simulink model "XFLUID02_reference"  (R2025a)
settings: Solver=ode23t  StartTime=0  StopTime=1.5  MaxStep=0.001  RelTol=1e-3  EnableMultiTasking=on
model workspace (MAT data in the model file):
  TRP_Par : object (value not decoded)
  fault_cylinder = 2
  inlet_area_factor = 1
  output_pressure_bar = 7
  pOutMeas_data = [7; 7]
  pOutMeas_time = [0; 1.5]
  pOut_Init_WKSP = 7
  pump_speed_rpm = 958
  seal_leak_fraction = 0
  speed_step_fraction = 0.08
  speed_step_time = 0.72
symbols that are objects in the model workspace (value not decoded): TRP_Par
undefined symbols (not defined in the file): Plunger, sm_pump_triplex_lib, smiData, X, Y, Z
libraries: sm_lib x133, fl_lib x62, nesl_utility x24, SimscapeFluids_lib x15, simulink x10, ee_lib x2
(part 5 of 7)

== system XFLUID02_reference/Pump/Plunger 1/Flow Out ==
  Gain : Gain  Gain=0.01/5
  Hydraulic Flow Rate Sensor : fl_lib/Isothermal Liquid/Sensors/Flow Rate Sensor (IL)  sensor_type=3
      settings: InternalSimscapePortConfiguration="{\"Bottom\":[],\"Left\":[{\"id\":\"A\",\"label\":\"A\",\"type\":\"foundation.isothermal_liquid.isothermal_liquid\"}],\"Right\":[{\"id\":\"B\",\"label\":\"B\",\"type\":\"foundation.isothermal_liquid.isothermal_liquid\"},{\"id\":\"M\",\"label\":\"M\",\"type\":\"output\"},{\"id\":\"V\",\"label\":\"V\",\"type\":\"output\"}],\"Top\":[]}"
      settings: LibrarySourceBlock=|
      | fl_lib/Hydraulic/Hydraulic Sensors/Hydraulic Flow Rate
      | Sensor
  Log_plunger1_flow : ToWorkspace  VariableName=plunger1_flow  SaveFormat=Timeseries  SampleTime=-1
  Lowpass Filter : TransferFcn  Denominator=[1/(2*pi*100) 1]
  PS Terminator : fl_lib/Physical Signals/Sinks/PS Terminator
  PS-Simulink Converter : nesl_utility/PS-Simulink Converter  PhysicalDomain=network_engine_domain  SubClassName=ps_output  LeftPortType=input  RightPortType=output  PseudoPeriodic=off  Frequencies=[]  VectorFormat=1-D array  Unit=lpm  AffineConversion=off
  Saturation : Saturate  UpperLimit=5  LowerLimit=0  ZeroCross=off
  A : PMIOPort  Side=Left
  B : PMIOPort  Port=2  Side=Right
  q : Outport  VectorParamsAs1DForOutWhenUnconnected=off
  wires:
  PS-Simulink Converter/1 -> Saturation/1, Log_plunger1_flow/1
  Saturation/1 -> Gain/1
  Gain/1 -> Lowpass Filter/1
  Lowpass Filter/1 -> q/1
  connections:
  PS Terminator/LConn1 -- Hydraulic Flow Rate Sensor/RConn2
  B/RConn1 -- Hydraulic Flow Rate Sensor/RConn1
  A/RConn1 -- Hydraulic Flow Rate Sensor/LConn1
  PS-Simulink Converter/LConn1 -- Hydraulic Flow Rate Sensor/RConn3

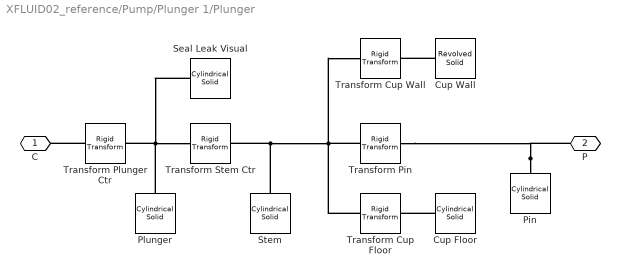
== system XFLUID02_reference/Pump/Plunger 1/Plunger ==
  Cup Floor : sm_lib/Body Elements/Cylindrical Solid  CylinderRadius=cup_rad_out-cup_thk  CylinderRadiusUnits=m  CylinderLength=cup_thk  CylinderLengthUnits=m  ExportEntireGeometry=off  InertiaType=CalculateFromGeometry  BasedOnType=Density  Density=plg_rho  DensityUnits=kg/m^3  Mass=1  MassUnits=kg  CenterOfMass=[0 0 0]  CenterOfMassUnits=m  MomentsOfInertia=[1 1 1]  MomentsOfInertiaUnits=kg*m^2  ProductsOfInertia=[1 1 1]  ProductsOfInertiaUnits=kg*m^2  GraphicType=FromGeometry  MarkerShape=Sphere  MarkerSize=10  GraphicVisPropType=SimpleVisualProperties  GraphicDiffuseColor=plg_clr  GraphicOpacity=plg_opc  GraphicSpecularColor=[0.5 0.5 0.5 1.0]  GraphicAmbientColor=[0.15 0.15 0.15 1.0]  GraphicEmissiveColor=[0.0 0.0 0.0 1.0]  GraphicShininess=75  DoExposeReferenceFrame=on  SerializedFrames=<Frames/>
  Cup Wall : sm_lib/Body Elements/Revolved Solid  RevolutionCrossSection=cup_xc_rev  RevolutionCrossSectionUnits=m  RevolutionExtent=Full  RevolutionAngle=180  RevolutionAngleUnits=deg  ExportConvexHullGeometry=off  InertiaType=CalculateFromGeometry  BasedOnType=Density  Density=plg_rho  DensityUnits=kg/m^3  Mass=1  MassUnits=kg  CenterOfMass=[0 0 0]  CenterOfMassUnits=m  MomentsOfInertia=[1 1 1]  MomentsOfInertiaUnits=kg*m^2  ProductsOfInertia=[1 1 1]  ProductsOfInertiaUnits=kg*m^2  GraphicType=FromGeometry  MarkerShape=Sphere  MarkerSize=10  GraphicVisPropType=SimpleVisualProperties  GraphicDiffuseColor=plg_clr  GraphicOpacity=plg_opc  GraphicSpecularColor=[0.5 0.5 0.5 1.0]  GraphicAmbientColor=[0.15 0.15 0.15 1.0]  GraphicEmissiveColor=[0.0 0.0 0.0 1.0]  GraphicShininess=75  DoExposeReferenceFrame=on  SerializedFrames=<Frames/>
  Pin : sm_lib/Body Elements/Cylindrical Solid  CylinderRadius=pin_rad  CylinderRadiusUnits=m  CylinderLength=pin_len  CylinderLengthUnits=m  ExportEntireGeometry=off  InertiaType=CalculateFromGeometry  BasedOnType=Density  Density=plg_rho  DensityUnits=kg/m^3  Mass=1  MassUnits=kg  CenterOfMass=[0 0 0]  CenterOfMassUnits=m  MomentsOfInertia=[1 1 1]  MomentsOfInertiaUnits=kg*m^2  ProductsOfInertia=[1 1 1]  ProductsOfInertiaUnits=kg*m^2  GraphicType=FromGeometry  MarkerShape=Sphere  MarkerSize=10  GraphicVisPropType=SimpleVisualProperties  GraphicDiffuseColor=conrod_clr*0.5  GraphicOpacity=conrod_opc  GraphicSpecularColor=[0.5 0.5 0.5 1.0]  GraphicAmbientColor=[0.15 0.15 0.15 1.0]  GraphicEmissiveColor=[0.0 0.0 0.0 1.0]  GraphicShininess=75  DoExposeReferenceFrame=on  SerializedFrames=<Frames/>
  Plunger : sm_lib/Body Elements/Cylindrical Solid  CylinderRadius=plgB_rad  CylinderRadiusUnits=m  CylinderLength=plgB_len  CylinderLengthUnits=m  ExportEntireGeometry=off  InertiaType=CalculateFromGeometry  BasedOnType=Density  Density=plg_rho  DensityUnits=kg/m^3  Mass=1  MassUnits=kg  CenterOfMass=[0 0 0]  CenterOfMassUnits=m  MomentsOfInertia=[1 1 1]  MomentsOfInertiaUnits=kg*m^2  ProductsOfInertia=[1 1 1]  ProductsOfInertiaUnits=kg*m^2  GraphicType=FromGeometry  MarkerShape=Sphere  MarkerSize=10  GraphicVisPropType=SimpleVisualProperties  GraphicDiffuseColor=plg_clr  GraphicOpacity=plg_opc  GraphicSpecularColor=[0.5 0.5 0.5 1.0]  GraphicAmbientColor=[0.15 0.15 0.15 1.0]  GraphicEmissiveColor=[0.0 0.0 0.0 1.0]  GraphicShininess=75  DoExposeReferenceFrame=on  SerializedFrames=<Frames/>
  Seal Leak Visual : sm_lib/Body Elements/Cylindrical Solid  CylinderRadius=seal_leak_vis_rad  CylinderRadiusUnits=m  CylinderLength=seal_leak_vis_len  CylinderLengthUnits=m  ExportEntireGeometry=off  InertiaType=CalculateFromGeometry  BasedOnType=Density  Density=0.0001  DensityUnits=kg/m^3  Mass=1  MassUnits=kg  CenterOfMass=[0 0 0]  CenterOfMassUnits=m  MomentsOfInertia=[1 1 1]  MomentsOfInertiaUnits=kg*m^2  ProductsOfInertia=[1 1 1]  ProductsOfInertiaUnits=kg*m^2  GraphicType=FromGeometry  MarkerShape=Sphere  MarkerSize=10  GraphicVisPropType=SimpleVisualProperties  GraphicDiffuseColor=seal_leak_vis_clr  GraphicOpacity=seal_leak_vis_opc  GraphicSpecularColor=[0.5 0.5 0.5 1.0]  GraphicAmbientColor=[0.15 0.15 0.15 1.0]  GraphicEmissiveColor=[0.0 0.0 0.0 1.0]  GraphicShininess=75  DoExposeReferenceFrame=on  SerializedFrames=<Frames/>
  Stem : sm_lib/Body Elements/Cylindrical Solid  CylinderRadius=stem_rad  CylinderRadiusUnits=m  CylinderLength=stem_len  CylinderLengthUnits=m  ExportEntireGeometry=off  InertiaType=CalculateFromGeometry  BasedOnType=Density  Density=plg_rho  DensityUnits=kg/m^3  Mass=1  MassUnits=kg  CenterOfMass=[0 0 0]  CenterOfMassUnits=m  MomentsOfInertia=[1 1 1]  MomentsOfInertiaUnits=kg*m^2  ProductsOfInertia=[1 1 1]  ProductsOfInertiaUnits=kg*m^2  GraphicType=FromGeometry  MarkerShape=Sphere  MarkerSize=10  GraphicVisPropType=SimpleVisualProperties  GraphicDiffuseColor=plg_clr  GraphicOpacity=plg_opc  GraphicSpecularColor=[0.5 0.5 0.5 1.0]  GraphicAmbientColor=[0.15 0.15 0.15 1.0]  GraphicEmissiveColor=[0.0 0.0 0.0 1.0]  GraphicShininess=75  DoExposeReferenceFrame=on  SerializedFrames=<Frames/>
  Transform Cup Floor : sm_lib/Frames and Transforms/Rigid Transform  RotationMethod=None  FollAlignAxisA=+X  BaseAlignAxisA=+Y  FollAlignAxisB=+Y  BaseAlignAxisB=+Z  RotationStandardAxis=+Z  RotationAngle=0.0  RotationAngleUnits=deg  RotationArbitraryAxis=[0 0 1]  RotationSequenceAxes=FollowerAxes  RotationSequence=XYX  RotationSequenceAngles=[0 0 0]  RotationSequenceAnglesUnits=deg  RotationMatrix=[1 0 0; 0 1 0; 0 0 1]  Quaternion=[1 0 0 0]  TranslationMethod=StandardAxis  TranslationCartesianOffset=[0 0 0]  TranslationCartesianOffsetUnits=m  TranslationStandardAxis=+Z  TranslationStandardOffset=stem_len/2+cup_thk/2  TranslationStandardOffsetUnits=m  TranslationROffset=0  TranslationROffsetUnits=m  TranslationThetaOffset=0  TranslationThetaOffsetUnits=deg  TranslationZOffset=0  TranslationZOffsetUnits=m
  Transform Cup Wall : sm_lib/Frames and Transforms/Rigid Transform  RotationMethod=None  FollAlignAxisA=+X  BaseAlignAxisA=+Y  FollAlignAxisB=+Y  BaseAlignAxisB=+Z  RotationStandardAxis=+Z  RotationAngle=0.0  RotationAngleUnits=deg  RotationArbitraryAxis=[0 0 1]  RotationSequenceAxes=FollowerAxes  RotationSequence=XYX  RotationSequenceAngles=[0 0 0]  RotationSequenceAnglesUnits=deg  RotationMatrix=[1 0 0; 0 1 0; 0 0 1]  Quaternion=[1 0 0 0]  TranslationMethod=StandardAxis  TranslationCartesianOffset=[0 0 0]  TranslationCartesianOffsetUnits=m  TranslationStandardAxis=+Z  TranslationStandardOffset=stem_len/2+cup_len/2  TranslationStandardOffsetUnits=m  TranslationROffset=0  TranslationROffsetUnits=m  TranslationThetaOffset=0  TranslationThetaOffsetUnits=deg  TranslationZOffset=0  TranslationZOffsetUnits=m
  Transform Plunger Ctr : sm_lib/Frames and Transforms/Rigid Transform  RotationMethod=None  FollAlignAxisA=+X  BaseAlignAxisA=+Y  FollAlignAxisB=+Y  BaseAlignAxisB=+Z  RotationStandardAxis=+Z  RotationAngle=0.0  RotationAngleUnits=deg  RotationArbitraryAxis=[0 0 1]  RotationSequenceAxes=FollowerAxes  RotationSequence=XYX  RotationSequenceAngles=[0 0 0]  RotationSequenceAnglesUnits=deg  RotationMatrix=[1 0 0; 0 1 0; 0 0 1]  Quaternion=[1 0 0 0]  TranslationMethod=StandardAxis  TranslationCartesianOffset=[0 0 0]  TranslationCartesianOffsetUnits=m  TranslationStandardAxis=+Z  TranslationStandardOffset=plgB_len/2  TranslationStandardOffsetUnits=m  TranslationROffset=0  TranslationROffsetUnits=m  TranslationThetaOffset=0  TranslationThetaOffsetUnits=deg  TranslationZOffset=0  TranslationZOffsetUnits=m
  Transform Stem Ctr : sm_lib/Frames and Transforms/Rigid Transform  RotationMethod=None  FollAlignAxisA=+X  BaseAlignAxisA=+Y  FollAlignAxisB=+Y  BaseAlignAxisB=+Z  RotationStandardAxis=+Z  RotationAngle=0.0  RotationAngleUnits=deg  RotationArbitraryAxis=[0 0 1]  RotationSequenceAxes=FollowerAxes  RotationSequence=XYX  RotationSequenceAngles=[0 0 0]  RotationSequenceAnglesUnits=deg  RotationMatrix=[1 0 0; 0 1 0; 0 0 1]  Quaternion=[1 0 0 0]  TranslationMethod=StandardAxis  TranslationCartesianOffset=[0 0 0]  TranslationCartesianOffsetUnits=m  TranslationStandardAxis=+Z  TranslationStandardOffset=plgB_len/2+stem_len/2  TranslationStandardOffsetUnits=m  TranslationROffset=0  TranslationROffsetUnits=m  TranslationThetaOffset=0  TranslationThetaOffsetUnits=deg  TranslationZOffset=0  TranslationZOffsetUnits=m
  Transform Pin : sm_lib/Frames and Transforms/Rigid Transform  RotationMethod=StandardAxis  FollAlignAxisA=+X  BaseAlignAxisA=+Y  FollAlignAxisB=+Y  BaseAlignAxisB=+Z  RotationStandardAxis=+Y  RotationAngle=90  RotationAngleUnits=deg  RotationArbitraryAxis=[0 0 1]  RotationSequenceAxes=FollowerAxes  RotationSequence=XYX  RotationSequenceAngles=[0 0 0]  RotationSequenceAnglesUnits=deg  RotationMatrix=[1 0 0; 0 1 0; 0 0 1]  Quaternion=[1 0 0 0]  TranslationMethod=StandardAxis  TranslationCartesianOffset=[0 0 0]  TranslationCartesianOffsetUnits=m  TranslationStandardAxis=+Z  TranslationStandardOffset=stem_len/2+cup_pinOffset  TranslationStandardOffsetUnits=m  TranslationROffset=0  TranslationROffsetUnits=m  TranslationThetaOffset=0  TranslationThetaOffsetUnits=deg  TranslationZOffset=0  TranslationZOffsetUnits=m
  C : PMIOPort  Side=Left
  P : PMIOPort  Port=2  Side=Right
  connections:
  Pin/RConn1 -- P/RConn1 -- Transform Pin/RConn1
  Cup Wall/RConn1 -- Transform Cup Wall/RConn1
  Cup Floor/RConn1 -- Transform Cup Floor/RConn1
  Plunger/RConn1 -- Transform Stem Ctr/LConn1 -- Seal Leak Visual/RConn1 -- Transform Plunger Ctr/RConn1
  Transform Plunger Ctr/LConn1 -- C/RConn1
  Stem/RConn1 -- Transform Cup Floor/LConn1 -- Transform Pin/LConn1 -- Transform Cup Wall/LConn1 -- Transform Stem Ctr/RConn1

== system XFLUID02_reference/Pump/Plunger 1/Rod ==
  Ring Pin : sm_lib/Body Elements/Revolved Solid  RevolutionCrossSection=conrod_ringP_xc_rev  RevolutionCrossSectionUnits=m  RevolutionExtent=Full  RevolutionAngle=180  RevolutionAngleUnits=deg  ExportConvexHullGeometry=off  InertiaType=CalculateFromGeometry  BasedOnType=Density  Density=conrod_rho  DensityUnits=kg/m^3  Mass=1  MassUnits=kg  CenterOfMass=[0 0 0]  CenterOfMassUnits=m  MomentsOfInertia=[1 1 1]  MomentsOfInertiaUnits=kg*m^2  ProductsOfInertia=[1 1 1]  ProductsOfInertiaUnits=kg*m^2  GraphicType=FromGeometry  MarkerShape=Sphere  MarkerSize=10  GraphicVisPropType=SimpleVisualProperties  GraphicDiffuseColor=conrod_clr  GraphicOpacity=conrod_opc  GraphicSpecularColor=[0.5 0.5 0.5 1.0]  GraphicAmbientColor=[0.15 0.15 0.15 1.0]  GraphicEmissiveColor=[0.0 0.0 0.0 1.0]  GraphicShininess=75  DoExposeReferenceFrame=on  SerializedFrames=<Frames/>
  Ring Shaft : sm_lib/Body Elements/Revolved Solid  RevolutionCrossSection=conrod_ringC_xc_rev  RevolutionCrossSectionUnits=m  RevolutionExtent=Full  RevolutionAngle=180  RevolutionAngleUnits=deg  ExportConvexHullGeometry=off  InertiaType=CalculateFromGeometry  BasedOnType=Density  Density=conrod_rho  DensityUnits=kg/m^3  Mass=1  MassUnits=kg  CenterOfMass=[0 0 0]  CenterOfMassUnits=m  MomentsOfInertia=[1 1 1]  MomentsOfInertiaUnits=kg*m^2  ProductsOfInertia=[1 1 1]  ProductsOfInertiaUnits=kg*m^2  GraphicType=FromGeometry  MarkerShape=Sphere  MarkerSize=10  GraphicVisPropType=SimpleVisualProperties  GraphicDiffuseColor=conrod_clr  GraphicOpacity=conrod_opc  GraphicSpecularColor=[0.5 0.5 0.5 1.0]  GraphicAmbientColor=[0.15 0.15 0.15 1.0]  GraphicEmissiveColor=[0.0 0.0 0.0 1.0]  GraphicShininess=75  DoExposeReferenceFrame=on  SerializedFrames=<Frames/>
  Transform Web Ctr : sm_lib/Frames and Transforms/Rigid Transform  RotationMethod=None  FollAlignAxisA=+X  BaseAlignAxisA=+Y  FollAlignAxisB=+Y  BaseAlignAxisB=+Z  RotationStandardAxis=+Z  RotationAngle=0.0  RotationAngleUnits=deg  RotationArbitraryAxis=[0 0 1]  RotationSequenceAxes=FollowerAxes  RotationSequence=XYX  RotationSequenceAngles=[0 0 0]  RotationSequenceAnglesUnits=deg  RotationMatrix=[1 0 0; 0 1 0; 0 0 1]  Quaternion=[1 0 0 0]  TranslationMethod=StandardAxis  TranslationCartesianOffset=[0 0 0]  TranslationCartesianOffsetUnits=m  TranslationStandardAxis=-X  TranslationStandardOffset=conrod_web_offP+conrod_web_len/2  TranslationStandardOffsetUnits=m  TranslationROffset=0  TranslationROffsetUnits=m  TranslationThetaOffset=0  TranslationThetaOffsetUnits=deg  TranslationZOffset=0  TranslationZOffsetUnits=m
  Transform Web RShaft : sm_lib/Frames and Transforms/Rigid Transform  RotationMethod=None  FollAlignAxisA=+X  BaseAlignAxisA=+Y  FollAlignAxisB=+Y  BaseAlignAxisB=+Z  RotationStandardAxis=+Z  RotationAngle=0.0  RotationAngleUnits=deg  RotationArbitraryAxis=[0 0 1]  RotationSequenceAxes=FollowerAxes  RotationSequence=XYX  RotationSequenceAngles=[0 0 0]  RotationSequenceAnglesUnits=deg  RotationMatrix=[1 0 0; 0 1 0; 0 0 1]  Quaternion=[1 0 0 0]  TranslationMethod=StandardAxis  TranslationCartesianOffset=[0 0 0]  TranslationCartesianOffsetUnits=m  TranslationStandardAxis=-X  TranslationStandardOffset=conrod_web_offC+conrod_web_len/2  TranslationStandardOffsetUnits=m  TranslationROffset=0  TranslationROffsetUnits=m  TranslationThetaOffset=0  TranslationThetaOffsetUnits=deg  TranslationZOffset=0  TranslationZOffsetUnits=m
  Web : sm_lib/Body Elements/Extruded Solid  ExtrusionType=General  PolygonNumSides=3  PolygonOuterRadius=1  PolygonOuterRadiusUnits=m  ExportEntireGeometry=off  ExtrusionCrossSection=conrod_web_xc  ExtrusionCrossSectionUnits=m  ExportConvexHullGeometry=off  ExtrusionLength=conrod_thk  ExtrusionLengthUnits=m  InertiaType=CalculateFromGeometry  BasedOnType=Density  Density=conrod_rho  DensityUnits=kg/m^3  Mass=1  MassUnits=kg  CenterOfMass=[0 0 0]  CenterOfMassUnits=m  MomentsOfInertia=[1 1 1]  MomentsOfInertiaUnits=kg*m^2  ProductsOfInertia=[1 1 1]  ProductsOfInertiaUnits=kg*m^2  GraphicType=FromGeometry  MarkerShape=Sphere  MarkerSize=10  GraphicVisPropType=SimpleVisualProperties  GraphicDiffuseColor=conrod_clr  GraphicOpacity=conrod_opc  GraphicSpecularColor=[0.5 0.5 0.5 1.0]  GraphicAmbientColor=[0.15 0.15 0.15 1.0]  GraphicEmissiveColor=[0.0 0.0 0.0 1.0]  GraphicShininess=75  DoExposeReferenceFrame=on  SerializedFrames=<Frames/>
  C : PMIOPort  Side=Left
  P : PMIOPort  Port=2  Side=Right
  connections:
  Transform Web Ctr/LConn1 -- Ring Pin/RConn1 -- C/RConn1
  Transform Web Ctr/RConn1 -- Transform Web RShaft/LConn1 -- Web/RConn1
  Ring Shaft/RConn1 -- P/RConn1 -- Transform Web RShaft/RConn1

== system XFLUID02_reference/Pump/Plunger 1/Seal Leak ==
  Off : Subsystem  VariantControl=Off
      mask Display: image('sm_pump_triplex_Seal_Leak_Off_IMAGE.png');
  On : Subsystem  VariantControl=On
      mask Display: image('sm_pump_triplex_Seal_Leak_On_IMAGE.png');
  Tune : Subsystem  VariantControl=Tune
      mask Display: image('sm_pump_triplex_Seal_Leak_On_IMAGE.png');
  " A " : PMIOPort  Side=Left

== system XFLUID02_reference/Pump/Plunger 1/Valve Visual ==
  "qi " : Inport
  "qo " : Inport  Port=2
  Off : Subsystem  VariantControl=Off
      mask Display: disp(' ');
  On : Subsystem  VariantControl=On
      mask Display: image('sm_pump_triplex_Valve_Vis_IMAGE.png');
  " W " : PMIOPort  Side=Right

== system XFLUID02_reference/Pump/Plunger 2/Cylinder ==
  Cylinder : sm_lib/Body Elements/Revolved Solid  RevolutionCrossSection=cyl_xc_rev  RevolutionCrossSectionUnits=m  RevolutionExtent=Full  RevolutionAngle=180  RevolutionAngleUnits=deg  ExportConvexHullGeometry=off  InertiaType=CalculateFromGeometry  BasedOnType=Density  Density=cyl_rho  DensityUnits=kg/m^3  Mass=1  MassUnits=kg  CenterOfMass=[0 0 0]  CenterOfMassUnits=m  MomentsOfInertia=[1 1 1]  MomentsOfInertiaUnits=kg*m^2  ProductsOfInertia=[1 1 1]  ProductsOfInertiaUnits=kg*m^2  GraphicType=FromGeometry  MarkerShape=Sphere  MarkerSize=10  GraphicVisPropType=SimpleVisualProperties  GraphicDiffuseColor=cyl_clr  GraphicOpacity=cyl_opc  GraphicSpecularColor=[0.5 0.5 0.5 1.0]  GraphicAmbientColor=[0.15 0.15 0.15 1.0]  GraphicEmissiveColor=[0.0 0.0 0.0 1.0]  GraphicShininess=75  DoExposeReferenceFrame=on  SerializedFrames=<Frames/>
  Obstruction Vis : sm_lib/Body Elements/Revolved Solid  RevolutionCrossSection=inlet_obstr_xc_rev  RevolutionCrossSectionUnits=m  RevolutionExtent=Full  RevolutionAngle=180  RevolutionAngleUnits=deg  ExportConvexHullGeometry=off  InertiaType=CalculateFromGeometry  BasedOnType=Density  Density=0.001  DensityUnits=kg/m^3  Mass=1  MassUnits=kg  CenterOfMass=[0 0 0]  CenterOfMassUnits=m  MomentsOfInertia=[1 1 1]  MomentsOfInertiaUnits=kg*m^2  ProductsOfInertia=[1 1 1]  ProductsOfInertiaUnits=kg*m^2  GraphicType=FromGeometry  MarkerShape=Sphere  MarkerSize=10  GraphicVisPropType=SimpleVisualProperties  GraphicDiffuseColor=inlet_obstr_clr  GraphicOpacity=inlet_obstr_opc  GraphicSpecularColor=[0.5 0.5 0.5 1.0]  GraphicAmbientColor=[0.15 0.15 0.15 1.0]  GraphicEmissiveColor=[0.0 0.0 0.0 1.0]  GraphicShininess=75  DoExposeReferenceFrame=on  SerializedFrames=<Frames/>
  Transform Ctr : sm_lib/Frames and Transforms/Rigid Transform  RotationMethod=None  FollAlignAxisA=+X  BaseAlignAxisA=+Y  FollAlignAxisB=+Y  BaseAlignAxisB=+Z  RotationStandardAxis=+Z  RotationAngle=0.0  RotationAngleUnits=deg  RotationArbitraryAxis=[0 0 1]  RotationSequenceAxes=FollowerAxes  RotationSequence=XYX  RotationSequenceAngles=[0 0 0]  RotationSequenceAnglesUnits=deg  RotationMatrix=[1 0 0; 0 1 0; 0 0 1]  Quaternion=[1 0 0 0]  TranslationMethod=StandardAxis  TranslationCartesianOffset=[0 0 0]  TranslationCartesianOffsetUnits=m  TranslationStandardAxis=+Z  TranslationStandardOffset=cyl_len/2  TranslationStandardOffsetUnits=m  TranslationROffset=0  TranslationROffsetUnits=m  TranslationThetaOffset=0  TranslationThetaOffsetUnits=deg  TranslationZOffset=0  TranslationZOffsetUnits=m
  Transform Manifold Opening : sm_lib/Frames and Transforms/Rigid Transform  RotationMethod=None  FollAlignAxisA=+X  BaseAlignAxisA=+Y  FollAlignAxisB=+Y  BaseAlignAxisB=+Z  RotationStandardAxis=+Z  RotationAngle=0.0  RotationAngleUnits=deg  RotationArbitraryAxis=[0 0 1]  RotationSequenceAxes=FollowerAxes  RotationSequence=XYX  RotationSequenceAngles=[0 0 0]  RotationSequenceAnglesUnits=deg  RotationMatrix=[1 0 0; 0 1 0; 0 0 1]  Quaternion=[1 0 0 0]  TranslationMethod=Cartesian  TranslationCartesianOffset=[0 -0.04 -0.045-0.005]  TranslationCartesianOffsetUnits=m  TranslationStandardAxis=+Z  TranslationStandardOffset=0  TranslationStandardOffsetUnits=m  TranslationROffset=0  TranslationROffsetUnits=m  TranslationThetaOffset=0  TranslationThetaOffsetUnits=deg  TranslationZOffset=0  TranslationZOffsetUnits=m
  W : PMIOPort  Side=Left
  P : PMIOPort  Port=2  Side=Right
  connections:
  Obstruction Vis/RConn1 -- Transform Manifold Opening/RConn1
  Cylinder/RConn1 -- Transform Ctr/RConn1
  Transform Ctr/LConn1 -- P/RConn1 -- Transform Manifold Opening/LConn1 -- W/RConn1

== system XFLUID02_reference/Pump/Plunger 2/Flow In ==
  Gain : Gain  Gain=0.01/5
  Hydraulic Flow Rate Sensor : fl_lib/Isothermal Liquid/Sensors/Flow Rate Sensor (IL)  sensor_type=3
      settings: InternalSimscapePortConfiguration="{\"Bottom\":[],\"Left\":[{\"id\":\"A\",\"label\":\"A\",\"type\":\"foundation.isothermal_liquid.isothermal_liquid\"}],\"Right\":[{\"id\":\"B\",\"label\":\"B\",\"type\":\"foundation.isothermal_liquid.isothermal_liquid\"},{\"id\":\"M\",\"label\":\"M\",\"type\":\"output\"},{\"id\":\"V\",\"label\":\"V\",\"type\":\"output\"}],\"Top\":[]}"
      settings: LibrarySourceBlock=|
      | fl_lib/Hydraulic/Hydraulic Sensors/Hydraulic Flow Rate
      | Sensor
  Lowpass Filter : TransferFcn  Denominator=[1/(2*pi*100) 1]
  PS Terminator : fl_lib/Physical Signals/Sinks/PS Terminator
  PS-Simulink Converter : nesl_utility/PS-Simulink Converter  PhysicalDomain=network_engine_domain  SubClassName=ps_output  LeftPortType=input  RightPortType=output  PseudoPeriodic=off  Frequencies=[]  VectorFormat=1-D array  Unit=lpm  AffineConversion=off
  Saturation : Saturate  UpperLimit=5  LowerLimit=0  ZeroCross=off
  B : PMIOPort  Side=Left
  A : PMIOPort  Port=2  Side=Right
  q : Outport  VectorParamsAs1DForOutWhenUnconnected=off
  wires:
  Lowpass Filter/1 -> q/1
  Gain/1 -> Lowpass Filter/1
  Saturation/1 -> Gain/1
  PS-Simulink Converter/1 -> Saturation/1
  connections:
  PS Terminator/LConn1 -- Hydraulic Flow Rate Sensor/RConn2
  B/RConn1 -- Hydraulic Flow Rate Sensor/RConn1
  A/RConn1 -- Hydraulic Flow Rate Sensor/LConn1
  PS-Simulink Converter/LConn1 -- Hydraulic Flow Rate Sensor/RConn3

== system XFLUID02_reference/Pump/Plunger 2/Flow Out ==
  Gain : Gain  Gain=0.01/5
  Hydraulic Flow Rate Sensor : fl_lib/Isothermal Liquid/Sensors/Flow Rate Sensor (IL)  sensor_type=3
      settings: InternalSimscapePortConfiguration="{\"Bottom\":[],\"Left\":[{\"id\":\"A\",\"label\":\"A\",\"type\":\"foundation.isothermal_liquid.isothermal_liquid\"}],\"Right\":[{\"id\":\"B\",\"label\":\"B\",\"type\":\"foundation.isothermal_liquid.isothermal_liquid\"},{\"id\":\"M\",\"label\":\"M\",\"type\":\"output\"},{\"id\":\"V\",\"label\":\"V\",\"type\":\"output\"}],\"Top\":[]}"
      settings: LibrarySourceBlock=|
      | fl_lib/Hydraulic/Hydraulic Sensors/Hydraulic Flow Rate
      | Sensor
  Log_plunger2_flow : ToWorkspace  VariableName=plunger2_flow  SaveFormat=Timeseries  SampleTime=-1
  Lowpass Filter : TransferFcn  Denominator=[1/(2*pi*100) 1]
  PS Terminator : fl_lib/Physical Signals/Sinks/PS Terminator
  PS-Simulink Converter : nesl_utility/PS-Simulink Converter  PhysicalDomain=network_engine_domain  SubClassName=ps_output  LeftPortType=input  RightPortType=output  PseudoPeriodic=off  Frequencies=[]  VectorFormat=1-D array  Unit=lpm  AffineConversion=off
  Saturation : Saturate  UpperLimit=5  LowerLimit=0  ZeroCross=off
  A : PMIOPort  Side=Left
  B : PMIOPort  Port=2  Side=Right
  q : Outport  VectorParamsAs1DForOutWhenUnconnected=off
  wires:
  PS-Simulink Converter/1 -> Saturation/1, Log_plunger2_flow/1
  Saturation/1 -> Gain/1
  Gain/1 -> Lowpass Filter/1
  Lowpass Filter/1 -> q/1
  connections:
  PS Terminator/LConn1 -- Hydraulic Flow Rate Sensor/RConn2
  B/RConn1 -- Hydraulic Flow Rate Sensor/RConn1
  A/RConn1 -- Hydraulic Flow Rate Sensor/LConn1
  PS-Simulink Converter/LConn1 -- Hydraulic Flow Rate Sensor/RConn3

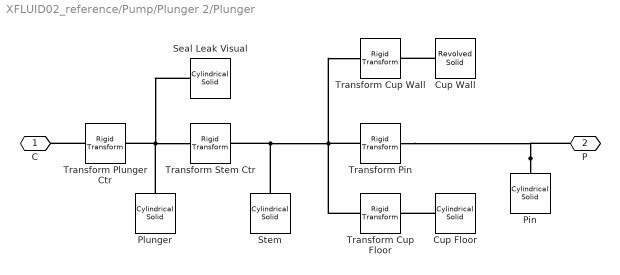
== system XFLUID02_reference/Pump/Plunger 2/Plunger ==
  Cup Floor : sm_lib/Body Elements/Cylindrical Solid  CylinderRadius=cup_rad_out-cup_thk  CylinderRadiusUnits=m  CylinderLength=cup_thk  CylinderLengthUnits=m  ExportEntireGeometry=off  InertiaType=CalculateFromGeometry  BasedOnType=Density  Density=plg_rho  DensityUnits=kg/m^3  Mass=1  MassUnits=kg  CenterOfMass=[0 0 0]  CenterOfMassUnits=m  MomentsOfInertia=[1 1 1]  MomentsOfInertiaUnits=kg*m^2  ProductsOfInertia=[1 1 1]  ProductsOfInertiaUnits=kg*m^2  GraphicType=FromGeometry  MarkerShape=Sphere  MarkerSize=10  GraphicVisPropType=SimpleVisualProperties  GraphicDiffuseColor=plg_clr  GraphicOpacity=plg_opc  GraphicSpecularColor=[0.5 0.5 0.5 1.0]  GraphicAmbientColor=[0.15 0.15 0.15 1.0]  GraphicEmissiveColor=[0.0 0.0 0.0 1.0]  GraphicShininess=75  DoExposeReferenceFrame=on  SerializedFrames=<Frames/>
  Cup Wall : sm_lib/Body Elements/Revolved Solid  RevolutionCrossSection=cup_xc_rev  RevolutionCrossSectionUnits=m  RevolutionExtent=Full  RevolutionAngle=180  RevolutionAngleUnits=deg  ExportConvexHullGeometry=off  InertiaType=CalculateFromGeometry  BasedOnType=Density  Density=plg_rho  DensityUnits=kg/m^3  Mass=1  MassUnits=kg  CenterOfMass=[0 0 0]  CenterOfMassUnits=m  MomentsOfInertia=[1 1 1]  MomentsOfInertiaUnits=kg*m^2  ProductsOfInertia=[1 1 1]  ProductsOfInertiaUnits=kg*m^2  GraphicType=FromGeometry  MarkerShape=Sphere  MarkerSize=10  GraphicVisPropType=SimpleVisualProperties  GraphicDiffuseColor=plg_clr  GraphicOpacity=plg_opc  GraphicSpecularColor=[0.5 0.5 0.5 1.0]  GraphicAmbientColor=[0.15 0.15 0.15 1.0]  GraphicEmissiveColor=[0.0 0.0 0.0 1.0]  GraphicShininess=75  DoExposeReferenceFrame=on  SerializedFrames=<Frames/>
  Pin : sm_lib/Body Elements/Cylindrical Solid  CylinderRadius=pin_rad  CylinderRadiusUnits=m  CylinderLength=pin_len  CylinderLengthUnits=m  ExportEntireGeometry=off  InertiaType=CalculateFromGeometry  BasedOnType=Density  Density=plg_rho  DensityUnits=kg/m^3  Mass=1  MassUnits=kg  CenterOfMass=[0 0 0]  CenterOfMassUnits=m  MomentsOfInertia=[1 1 1]  MomentsOfInertiaUnits=kg*m^2  ProductsOfInertia=[1 1 1]  ProductsOfInertiaUnits=kg*m^2  GraphicType=FromGeometry  MarkerShape=Sphere  MarkerSize=10  GraphicVisPropType=SimpleVisualProperties  GraphicDiffuseColor=conrod_clr*0.5  GraphicOpacity=conrod_opc  GraphicSpecularColor=[0.5 0.5 0.5 1.0]  GraphicAmbientColor=[0.15 0.15 0.15 1.0]  GraphicEmissiveColor=[0.0 0.0 0.0 1.0]  GraphicShininess=75  DoExposeReferenceFrame=on  SerializedFrames=<Frames/>
  Plunger : sm_lib/Body Elements/Cylindrical Solid  CylinderRadius=plgB_rad  CylinderRadiusUnits=m  CylinderLength=plgB_len  CylinderLengthUnits=m  ExportEntireGeometry=off  InertiaType=CalculateFromGeometry  BasedOnType=Density  Density=plg_rho  DensityUnits=kg/m^3  Mass=1  MassUnits=kg  CenterOfMass=[0 0 0]  CenterOfMassUnits=m  MomentsOfInertia=[1 1 1]  MomentsOfInertiaUnits=kg*m^2  ProductsOfInertia=[1 1 1]  ProductsOfInertiaUnits=kg*m^2  GraphicType=FromGeometry  MarkerShape=Sphere  MarkerSize=10  GraphicVisPropType=SimpleVisualProperties  GraphicDiffuseColor=plg_clr  GraphicOpacity=plg_opc  GraphicSpecularColor=[0.5 0.5 0.5 1.0]  GraphicAmbientColor=[0.15 0.15 0.15 1.0]  GraphicEmissiveColor=[0.0 0.0 0.0 1.0]  GraphicShininess=75  DoExposeReferenceFrame=on  SerializedFrames=<Frames/>
  Seal Leak Visual : sm_lib/Body Elements/Cylindrical Solid  CylinderRadius=seal_leak_vis_rad  CylinderRadiusUnits=m  CylinderLength=seal_leak_vis_len  CylinderLengthUnits=m  ExportEntireGeometry=off  InertiaType=CalculateFromGeometry  BasedOnType=Density  Density=0.0001  DensityUnits=kg/m^3  Mass=1  MassUnits=kg  CenterOfMass=[0 0 0]  CenterOfMassUnits=m  MomentsOfInertia=[1 1 1]  MomentsOfInertiaUnits=kg*m^2  ProductsOfInertia=[1 1 1]  ProductsOfInertiaUnits=kg*m^2  GraphicType=FromGeometry  MarkerShape=Sphere  MarkerSize=10  GraphicVisPropType=SimpleVisualProperties  GraphicDiffuseColor=seal_leak_vis_clr  GraphicOpacity=seal_leak_vis_opc  GraphicSpecularColor=[0.5 0.5 0.5 1.0]  GraphicAmbientColor=[0.15 0.15 0.15 1.0]  GraphicEmissiveColor=[0.0 0.0 0.0 1.0]  GraphicShininess=75  DoExposeReferenceFrame=on  SerializedFrames=<Frames/>
  Stem : sm_lib/Body Elements/Cylindrical Solid  CylinderRadius=stem_rad  CylinderRadiusUnits=m  CylinderLength=stem_len  CylinderLengthUnits=m  ExportEntireGeometry=off  InertiaType=CalculateFromGeometry  BasedOnType=Density  Density=plg_rho  DensityUnits=kg/m^3  Mass=1  MassUnits=kg  CenterOfMass=[0 0 0]  CenterOfMassUnits=m  MomentsOfInertia=[1 1 1]  MomentsOfInertiaUnits=kg*m^2  ProductsOfInertia=[1 1 1]  ProductsOfInertiaUnits=kg*m^2  GraphicType=FromGeometry  MarkerShape=Sphere  MarkerSize=10  GraphicVisPropType=SimpleVisualProperties  GraphicDiffuseColor=plg_clr  GraphicOpacity=plg_opc  GraphicSpecularColor=[0.5 0.5 0.5 1.0]  GraphicAmbientColor=[0.15 0.15 0.15 1.0]  GraphicEmissiveColor=[0.0 0.0 0.0 1.0]  GraphicShininess=75  DoExposeReferenceFrame=on  SerializedFrames=<Frames/>
  Transform Cup Floor : sm_lib/Frames and Transforms/Rigid Transform  RotationMethod=None  FollAlignAxisA=+X  BaseAlignAxisA=+Y  FollAlignAxisB=+Y  BaseAlignAxisB=+Z  RotationStandardAxis=+Z  RotationAngle=0.0  RotationAngleUnits=deg  RotationArbitraryAxis=[0 0 1]  RotationSequenceAxes=FollowerAxes  RotationSequence=XYX  RotationSequenceAngles=[0 0 0]  RotationSequenceAnglesUnits=deg  RotationMatrix=[1 0 0; 0 1 0; 0 0 1]  Quaternion=[1 0 0 0]  TranslationMethod=StandardAxis  TranslationCartesianOffset=[0 0 0]  TranslationCartesianOffsetUnits=m  TranslationStandardAxis=+Z  TranslationStandardOffset=stem_len/2+cup_thk/2  TranslationStandardOffsetUnits=m  TranslationROffset=0  TranslationROffsetUnits=m  TranslationThetaOffset=0  TranslationThetaOffsetUnits=deg  TranslationZOffset=0  TranslationZOffsetUnits=m
  Transform Cup Wall : sm_lib/Frames and Transforms/Rigid Transform  RotationMethod=None  FollAlignAxisA=+X  BaseAlignAxisA=+Y  FollAlignAxisB=+Y  BaseAlignAxisB=+Z  RotationStandardAxis=+Z  RotationAngle=0.0  RotationAngleUnits=deg  RotationArbitraryAxis=[0 0 1]  RotationSequenceAxes=FollowerAxes  RotationSequence=XYX  RotationSequenceAngles=[0 0 0]  RotationSequenceAnglesUnits=deg  RotationMatrix=[1 0 0; 0 1 0; 0 0 1]  Quaternion=[1 0 0 0]  TranslationMethod=StandardAxis  TranslationCartesianOffset=[0 0 0]  TranslationCartesianOffsetUnits=m  TranslationStandardAxis=+Z  TranslationStandardOffset=stem_len/2+cup_len/2  TranslationStandardOffsetUnits=m  TranslationROffset=0  TranslationROffsetUnits=m  TranslationThetaOffset=0  TranslationThetaOffsetUnits=deg  TranslationZOffset=0  TranslationZOffsetUnits=m
  Transform Plunger Ctr : sm_lib/Frames and Transforms/Rigid Transform  RotationMethod=None  FollAlignAxisA=+X  BaseAlignAxisA=+Y  FollAlignAxisB=+Y  BaseAlignAxisB=+Z  RotationStandardAxis=+Z  RotationAngle=0.0  RotationAngleUnits=deg  RotationArbitraryAxis=[0 0 1]  RotationSequenceAxes=FollowerAxes  RotationSequence=XYX  RotationSequenceAngles=[0 0 0]  RotationSequenceAnglesUnits=deg  RotationMatrix=[1 0 0; 0 1 0; 0 0 1]  Quaternion=[1 0 0 0]  TranslationMethod=StandardAxis  TranslationCartesianOffset=[0 0 0]  TranslationCartesianOffsetUnits=m  TranslationStandardAxis=+Z  TranslationStandardOffset=plgB_len/2  TranslationStandardOffsetUnits=m  TranslationROffset=0  TranslationROffsetUnits=m  TranslationThetaOffset=0  TranslationThetaOffsetUnits=deg  TranslationZOffset=0  TranslationZOffsetUnits=m
  Transform Stem Ctr : sm_lib/Frames and Transforms/Rigid Transform  RotationMethod=None  FollAlignAxisA=+X  BaseAlignAxisA=+Y  FollAlignAxisB=+Y  BaseAlignAxisB=+Z  RotationStandardAxis=+Z  RotationAngle=0.0  RotationAngleUnits=deg  RotationArbitraryAxis=[0 0 1]  RotationSequenceAxes=FollowerAxes  RotationSequence=XYX  RotationSequenceAngles=[0 0 0]  RotationSequenceAnglesUnits=deg  RotationMatrix=[1 0 0; 0 1 0; 0 0 1]  Quaternion=[1 0 0 0]  TranslationMethod=StandardAxis  TranslationCartesianOffset=[0 0 0]  TranslationCartesianOffsetUnits=m  TranslationStandardAxis=+Z  TranslationStandardOffset=plgB_len/2+stem_len/2  TranslationStandardOffsetUnits=m  TranslationROffset=0  TranslationROffsetUnits=m  TranslationThetaOffset=0  TranslationThetaOffsetUnits=deg  TranslationZOffset=0  TranslationZOffsetUnits=m
  Transform Pin : sm_lib/Frames and Transforms/Rigid Transform  RotationMethod=StandardAxis  FollAlignAxisA=+X  BaseAlignAxisA=+Y  FollAlignAxisB=+Y  BaseAlignAxisB=+Z  RotationStandardAxis=+Y  RotationAngle=90  RotationAngleUnits=deg  RotationArbitraryAxis=[0 0 1]  RotationSequenceAxes=FollowerAxes  RotationSequence=XYX  RotationSequenceAngles=[0 0 0]  RotationSequenceAnglesUnits=deg  RotationMatrix=[1 0 0; 0 1 0; 0 0 1]  Quaternion=[1 0 0 0]  TranslationMethod=StandardAxis  TranslationCartesianOffset=[0 0 0]  TranslationCartesianOffsetUnits=m  TranslationStandardAxis=+Z  TranslationStandardOffset=stem_len/2+cup_pinOffset  TranslationStandardOffsetUnits=m  TranslationROffset=0  TranslationROffsetUnits=m  TranslationThetaOffset=0  TranslationThetaOffsetUnits=deg  TranslationZOffset=0  TranslationZOffsetUnits=m
  C : PMIOPort  Side=Left
  P : PMIOPort  Port=2  Side=Right
  connections:
  Pin/RConn1 -- P/RConn1 -- Transform Pin/RConn1
  Cup Wall/RConn1 -- Transform Cup Wall/RConn1
  Cup Floor/RConn1 -- Transform Cup Floor/RConn1
  Plunger/RConn1 -- Transform Stem Ctr/LConn1 -- Seal Leak Visual/RConn1 -- Transform Plunger Ctr/RConn1
  Transform Plunger Ctr/LConn1 -- C/RConn1
  Stem/RConn1 -- Transform Cup Floor/LConn1 -- Transform Pin/LConn1 -- Transform Cup Wall/LConn1 -- Transform Stem Ctr/RConn1

== system XFLUID02_reference/Pump/Plunger 2/Rod ==
  Ring Pin : sm_lib/Body Elements/Revolved Solid  RevolutionCrossSection=conrod_ringP_xc_rev  RevolutionCrossSectionUnits=m  RevolutionExtent=Full  RevolutionAngle=180  RevolutionAngleUnits=deg  ExportConvexHullGeometry=off  InertiaType=CalculateFromGeometry  BasedOnType=Density  Density=conrod_rho  DensityUnits=kg/m^3  Mass=1  MassUnits=kg  CenterOfMass=[0 0 0]  CenterOfMassUnits=m  MomentsOfInertia=[1 1 1]  MomentsOfInertiaUnits=kg*m^2  ProductsOfInertia=[1 1 1]  ProductsOfInertiaUnits=kg*m^2  GraphicType=FromGeometry  MarkerShape=Sphere  MarkerSize=10  GraphicVisPropType=SimpleVisualProperties  GraphicDiffuseColor=conrod_clr  GraphicOpacity=conrod_opc  GraphicSpecularColor=[0.5 0.5 0.5 1.0]  GraphicAmbientColor=[0.15 0.15 0.15 1.0]  GraphicEmissiveColor=[0.0 0.0 0.0 1.0]  GraphicShininess=75  DoExposeReferenceFrame=on  SerializedFrames=<Frames/>
  Ring Shaft : sm_lib/Body Elements/Revolved Solid  RevolutionCrossSection=conrod_ringC_xc_rev  RevolutionCrossSectionUnits=m  RevolutionExtent=Full  RevolutionAngle=180  RevolutionAngleUnits=deg  ExportConvexHullGeometry=off  InertiaType=CalculateFromGeometry  BasedOnType=Density  Density=conrod_rho  DensityUnits=kg/m^3  Mass=1  MassUnits=kg  CenterOfMass=[0 0 0]  CenterOfMassUnits=m  MomentsOfInertia=[1 1 1]  MomentsOfInertiaUnits=kg*m^2  ProductsOfInertia=[1 1 1]  ProductsOfInertiaUnits=kg*m^2  GraphicType=FromGeometry  MarkerShape=Sphere  MarkerSize=10  GraphicVisPropType=SimpleVisualProperties  GraphicDiffuseColor=conrod_clr  GraphicOpacity=conrod_opc  GraphicSpecularColor=[0.5 0.5 0.5 1.0]  GraphicAmbientColor=[0.15 0.15 0.15 1.0]  GraphicEmissiveColor=[0.0 0.0 0.0 1.0]  GraphicShininess=75  DoExposeReferenceFrame=on  SerializedFrames=<Frames/>
  Transform Web Ctr : sm_lib/Frames and Transforms/Rigid Transform  RotationMethod=None  FollAlignAxisA=+X  BaseAlignAxisA=+Y  FollAlignAxisB=+Y  BaseAlignAxisB=+Z  RotationStandardAxis=+Z  RotationAngle=0.0  RotationAngleUnits=deg  RotationArbitraryAxis=[0 0 1]  RotationSequenceAxes=FollowerAxes  RotationSequence=XYX  RotationSequenceAngles=[0 0 0]  RotationSequenceAnglesUnits=deg  RotationMatrix=[1 0 0; 0 1 0; 0 0 1]  Quaternion=[1 0 0 0]  TranslationMethod=StandardAxis  TranslationCartesianOffset=[0 0 0]  TranslationCartesianOffsetUnits=m  TranslationStandardAxis=-X  TranslationStandardOffset=conrod_web_offP+conrod_web_len/2  TranslationStandardOffsetUnits=m  TranslationROffset=0  TranslationROffsetUnits=m  TranslationThetaOffset=0  TranslationThetaOffsetUnits=deg  TranslationZOffset=0  TranslationZOffsetUnits=m
  Transform Web RShaft : sm_lib/Frames and Transforms/Rigid Transform  RotationMethod=None  FollAlignAxisA=+X  BaseAlignAxisA=+Y  FollAlignAxisB=+Y  BaseAlignAxisB=+Z  RotationStandardAxis=+Z  RotationAngle=0.0  RotationAngleUnits=deg  RotationArbitraryAxis=[0 0 1]  RotationSequenceAxes=FollowerAxes  RotationSequence=XYX  RotationSequenceAngles=[0 0 0]  RotationSequenceAnglesUnits=deg  RotationMatrix=[1 0 0; 0 1 0; 0 0 1]  Quaternion=[1 0 0 0]  TranslationMethod=StandardAxis  TranslationCartesianOffset=[0 0 0]  TranslationCartesianOffsetUnits=m  TranslationStandardAxis=-X  TranslationStandardOffset=conrod_web_offC+conrod_web_len/2  TranslationStandardOffsetUnits=m  TranslationROffset=0  TranslationROffsetUnits=m  TranslationThetaOffset=0  TranslationThetaOffsetUnits=deg  TranslationZOffset=0  TranslationZOffsetUnits=m
  Web : sm_lib/Body Elements/Extruded Solid  ExtrusionType=General  PolygonNumSides=3  PolygonOuterRadius=1  PolygonOuterRadiusUnits=m  ExportEntireGeometry=off  ExtrusionCrossSection=conrod_web_xc  ExtrusionCrossSectionUnits=m  ExportConvexHullGeometry=off  ExtrusionLength=conrod_thk  ExtrusionLengthUnits=m  InertiaType=CalculateFromGeometry  BasedOnType=Density  Density=conrod_rho  DensityUnits=kg/m^3  Mass=1  MassUnits=kg  CenterOfMass=[0 0 0]  CenterOfMassUnits=m  MomentsOfInertia=[1 1 1]  MomentsOfInertiaUnits=kg*m^2  ProductsOfInertia=[1 1 1]  ProductsOfInertiaUnits=kg*m^2  GraphicType=FromGeometry  MarkerShape=Sphere  MarkerSize=10  GraphicVisPropType=SimpleVisualProperties  GraphicDiffuseColor=conrod_clr  GraphicOpacity=conrod_opc  GraphicSpecularColor=[0.5 0.5 0.5 1.0]  GraphicAmbientColor=[0.15 0.15 0.15 1.0]  GraphicEmissiveColor=[0.0 0.0 0.0 1.0]  GraphicShininess=75  DoExposeReferenceFrame=on  SerializedFrames=<Frames/>
  C : PMIOPort  Side=Left
  P : PMIOPort  Port=2  Side=Right
  connections:
  Transform Web Ctr/LConn1 -- Ring Pin/RConn1 -- C/RConn1
  Transform Web Ctr/RConn1 -- Transform Web RShaft/LConn1 -- Web/RConn1
  Ring Shaft/RConn1 -- P/RConn1 -- Transform Web RShaft/RConn1

== system XFLUID02_reference/Pump/Plunger 2/Seal Leak ==
  Off : Subsystem  VariantControl=Off
      mask Display: image('sm_pump_triplex_Seal_Leak_Off_IMAGE.png');
  On : Subsystem  VariantControl=On
      mask Display: image('sm_pump_triplex_Seal_Leak_On_IMAGE.png');
  Tune : Subsystem  VariantControl=Tune
      mask Display: image('sm_pump_triplex_Seal_Leak_On_IMAGE.png');
  " A " : PMIOPort  Side=Left

== system XFLUID02_reference/Pump/Plunger 2/Valve Visual ==
  "qi " : Inport
  "qo " : Inport  Port=2
  Off : Subsystem  VariantControl=Off
      mask Display: disp(' ');
  On : Subsystem  VariantControl=On
      mask Display: image('sm_pump_triplex_Valve_Vis_IMAGE.png');
  " W " : PMIOPort  Side=Right

== system XFLUID02_reference/Pump/Plunger 3/Cylinder ==
  Cylinder : sm_lib/Body Elements/Revolved Solid  RevolutionCrossSection=cyl_xc_rev  RevolutionCrossSectionUnits=m  RevolutionExtent=Full  RevolutionAngle=180  RevolutionAngleUnits=deg  ExportConvexHullGeometry=off  InertiaType=CalculateFromGeometry  BasedOnType=Density  Density=cyl_rho  DensityUnits=kg/m^3  Mass=1  MassUnits=kg  CenterOfMass=[0 0 0]  CenterOfMassUnits=m  MomentsOfInertia=[1 1 1]  MomentsOfInertiaUnits=kg*m^2  ProductsOfInertia=[1 1 1]  ProductsOfInertiaUnits=kg*m^2  GraphicType=FromGeometry  MarkerShape=Sphere  MarkerSize=10  GraphicVisPropType=SimpleVisualProperties  GraphicDiffuseColor=cyl_clr  GraphicOpacity=cyl_opc  GraphicSpecularColor=[0.5 0.5 0.5 1.0]  GraphicAmbientColor=[0.15 0.15 0.15 1.0]  GraphicEmissiveColor=[0.0 0.0 0.0 1.0]  GraphicShininess=75  DoExposeReferenceFrame=on  SerializedFrames=<Frames/>
  Obstruction Vis : sm_lib/Body Elements/Revolved Solid  RevolutionCrossSection=inlet_obstr_xc_rev  RevolutionCrossSectionUnits=m  RevolutionExtent=Full  RevolutionAngle=180  RevolutionAngleUnits=deg  ExportConvexHullGeometry=off  InertiaType=CalculateFromGeometry  BasedOnType=Density  Density=0.001  DensityUnits=kg/m^3  Mass=1  MassUnits=kg  CenterOfMass=[0 0 0]  CenterOfMassUnits=m  MomentsOfInertia=[1 1 1]  MomentsOfInertiaUnits=kg*m^2  ProductsOfInertia=[1 1 1]  ProductsOfInertiaUnits=kg*m^2  GraphicType=FromGeometry  MarkerShape=Sphere  MarkerSize=10  GraphicVisPropType=SimpleVisualProperties  GraphicDiffuseColor=inlet_obstr_clr  GraphicOpacity=inlet_obstr_opc  GraphicSpecularColor=[0.5 0.5 0.5 1.0]  GraphicAmbientColor=[0.15 0.15 0.15 1.0]  GraphicEmissiveColor=[0.0 0.0 0.0 1.0]  GraphicShininess=75  DoExposeReferenceFrame=on  SerializedFrames=<Frames/>
  Transform Ctr : sm_lib/Frames and Transforms/Rigid Transform  RotationMethod=None  FollAlignAxisA=+X  BaseAlignAxisA=+Y  FollAlignAxisB=+Y  BaseAlignAxisB=+Z  RotationStandardAxis=+Z  RotationAngle=0.0  RotationAngleUnits=deg  RotationArbitraryAxis=[0 0 1]  RotationSequenceAxes=FollowerAxes  RotationSequence=XYX  RotationSequenceAngles=[0 0 0]  RotationSequenceAnglesUnits=deg  RotationMatrix=[1 0 0; 0 1 0; 0 0 1]  Quaternion=[1 0 0 0]  TranslationMethod=StandardAxis  TranslationCartesianOffset=[0 0 0]  TranslationCartesianOffsetUnits=m  TranslationStandardAxis=+Z  TranslationStandardOffset=cyl_len/2  TranslationStandardOffsetUnits=m  TranslationROffset=0  TranslationROffsetUnits=m  TranslationThetaOffset=0  TranslationThetaOffsetUnits=deg  TranslationZOffset=0  TranslationZOffsetUnits=m
  Transform Manifold Opening : sm_lib/Frames and Transforms/Rigid Transform  RotationMethod=None  FollAlignAxisA=+X  BaseAlignAxisA=+Y  FollAlignAxisB=+Y  BaseAlignAxisB=+Z  RotationStandardAxis=+Z  RotationAngle=0.0  RotationAngleUnits=deg  RotationArbitraryAxis=[0 0 1]  RotationSequenceAxes=FollowerAxes  RotationSequence=XYX  RotationSequenceAngles=[0 0 0]  RotationSequenceAnglesUnits=deg  RotationMatrix=[1 0 0; 0 1 0; 0 0 1]  Quaternion=[1 0 0 0]  TranslationMethod=Cartesian  TranslationCartesianOffset=[0 -0.04 -0.045-0.005]  TranslationCartesianOffsetUnits=m  TranslationStandardAxis=+Z  TranslationStandardOffset=0  TranslationStandardOffsetUnits=m  TranslationROffset=0  TranslationROffsetUnits=m  TranslationThetaOffset=0  TranslationThetaOffsetUnits=deg  TranslationZOffset=0  TranslationZOffsetUnits=m
  W : PMIOPort  Side=Left
  P : PMIOPort  Port=2  Side=Right
  connections:
  Obstruction Vis/RConn1 -- Transform Manifold Opening/RConn1
  Cylinder/RConn1 -- Transform Ctr/RConn1
  Transform Ctr/LConn1 -- P/RConn1 -- Transform Manifold Opening/LConn1 -- W/RConn1

== system XFLUID02_reference/Pump/Plunger 3/Flow In ==
  Gain : Gain  Gain=0.01/5
  Hydraulic Flow Rate Sensor : fl_lib/Isothermal Liquid/Sensors/Flow Rate Sensor (IL)  sensor_type=3
      settings: InternalSimscapePortConfiguration="{\"Bottom\":[],\"Left\":[{\"id\":\"A\",\"label\":\"A\",\"type\":\"foundation.isothermal_liquid.isothermal_liquid\"}],\"Right\":[{\"id\":\"B\",\"label\":\"B\",\"type\":\"foundation.isothermal_liquid.isothermal_liquid\"},{\"id\":\"M\",\"label\":\"M\",\"type\":\"output\"},{\"id\":\"V\",\"label\":\"V\",\"type\":\"output\"}],\"Top\":[]}"
      settings: LibrarySourceBlock=|
      | fl_lib/Hydraulic/Hydraulic Sensors/Hydraulic Flow Rate
      | Sensor
  Lowpass Filter : TransferFcn  Denominator=[1/(2*pi*100) 1]
  PS Terminator : fl_lib/Physical Signals/Sinks/PS Terminator
  PS-Simulink Converter : nesl_utility/PS-Simulink Converter  PhysicalDomain=network_engine_domain  SubClassName=ps_output  LeftPortType=input  RightPortType=output  PseudoPeriodic=off  Frequencies=[]  VectorFormat=1-D array  Unit=lpm  AffineConversion=off
  Saturation : Saturate  UpperLimit=5  LowerLimit=0  ZeroCross=off
  B : PMIOPort  Side=Left
  A : PMIOPort  Port=2  Side=Right
  q : Outport  VectorParamsAs1DForOutWhenUnconnected=off
  wires:
  Lowpass Filter/1 -> q/1
  Gain/1 -> Lowpass Filter/1
  Saturation/1 -> Gain/1
  PS-Simulink Converter/1 -> Saturation/1
  connections:
  PS Terminator/LConn1 -- Hydraulic Flow Rate Sensor/RConn2
  B/RConn1 -- Hydraulic Flow Rate Sensor/RConn1
  A/RConn1 -- Hydraulic Flow Rate Sensor/LConn1
  PS-Simulink Converter/LConn1 -- Hydraulic Flow Rate Sensor/RConn3

== system XFLUID02_reference/Pump/Plunger 3/Flow Out ==
  Gain : Gain  Gain=0.01/5
  Hydraulic Flow Rate Sensor : fl_lib/Isothermal Liquid/Sensors/Flow Rate Sensor (IL)  sensor_type=3
      settings: InternalSimscapePortConfiguration="{\"Bottom\":[],\"Left\":[{\"id\":\"A\",\"label\":\"A\",\"type\":\"foundation.isothermal_liquid.isothermal_liquid\"}],\"Right\":[{\"id\":\"B\",\"label\":\"B\",\"type\":\"foundation.isothermal_liquid.isothermal_liquid\"},{\"id\":\"M\",\"label\":\"M\",\"type\":\"output\"},{\"id\":\"V\",\"label\":\"V\",\"type\":\"output\"}],\"Top\":[]}"
      settings: LibrarySourceBlock=|
      | fl_lib/Hydraulic/Hydraulic Sensors/Hydraulic Flow Rate
      | Sensor
  Log_plunger3_flow : ToWorkspace  VariableName=plunger3_flow  SaveFormat=Timeseries  SampleTime=-1
  Lowpass Filter : TransferFcn  Denominator=[1/(2*pi*100) 1]
  PS Terminator : fl_lib/Physical Signals/Sinks/PS Terminator
  PS-Simulink Converter : nesl_utility/PS-Simulink Converter  PhysicalDomain=network_engine_domain  SubClassName=ps_output  LeftPortType=input  RightPortType=output  PseudoPeriodic=off  Frequencies=[]  VectorFormat=1-D array  Unit=lpm  AffineConversion=off
  Saturation : Saturate  UpperLimit=5  LowerLimit=0  ZeroCross=off
  A : PMIOPort  Side=Left
  B : PMIOPort  Port=2  Side=Right
  q : Outport  VectorParamsAs1DForOutWhenUnconnected=off
  wires:
  PS-Simulink Converter/1 -> Saturation/1, Log_plunger3_flow/1
  Saturation/1 -> Gain/1
  Gain/1 -> Lowpass Filter/1
  Lowpass Filter/1 -> q/1
  connections:
  PS Terminator/LConn1 -- Hydraulic Flow Rate Sensor/RConn2
  B/RConn1 -- Hydraulic Flow Rate Sensor/RConn1
  A/RConn1 -- Hydraulic Flow Rate Sensor/LConn1
  PS-Simulink Converter/LConn1 -- Hydraulic Flow Rate Sensor/RConn3
